simulink library "sm_wheel_loader_lib"  (R2025a)
settings: Solver=VariableStepAuto  StartTime=0.0  StopTime=10.0  RelTol=1e-3
undefined symbols (not defined in the file): AToTOrificeVector, BiPOrificeVector, boomHEArea, boomREArea, BToTOrificeVector, fluids, GRake, GToothL, GToothR, HMPST, HydFcnParams, logLoad, Position, PToAOrificeVector, PToBOrificeVector, RakeL, RakeR, testInput, Wheel_Loader, X, Y, Z
libraries: sm_lib x694, fl_lib x183, nesl_utility x74, SimscapeFluids_lib x62, sdl_lib x25, cvt_components_lib x25, simulink_extras x5, $bdroot x4, wheel_loader_contact_lib x4, ee_lib x2, SignalEditorBlockLib x1, batteryecm_lib x1
(part 4 of 26)

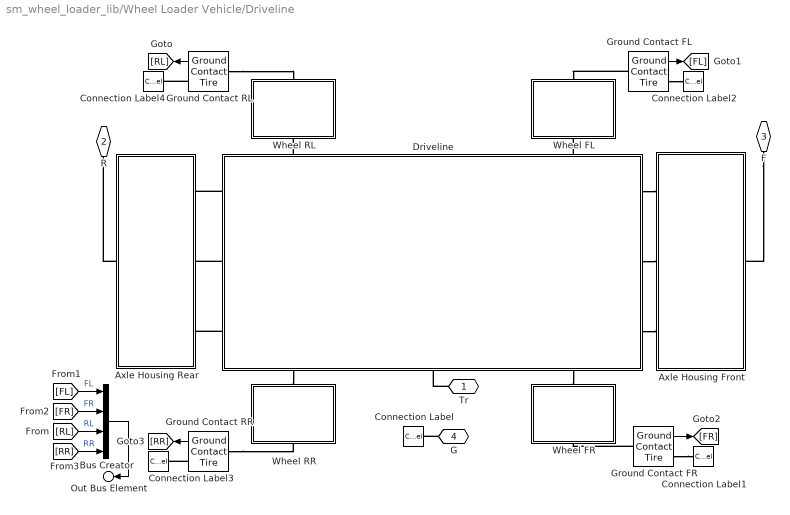
== system sm_wheel_loader_lib/Wheel Loader Vehicle/Driveline ==
  Axle Housing Front : Subsystem  Tag=26328293-4415-CB41-A9FB-B9AA4EE664BB  mask{fa_casing_opc=HMPST.Vis.FAxleHou.opc}
      mask prompts: fa_casing_opc "Casing Opacity"
      mask Display: image('sm_wheel_loader_Driveline3D_FAxleHou_IMAGE.png')
  Axle Housing Rear : Subsystem  Tag=1D918CE5-F562-3F48-9394-464191D609BF  mask{ra_casing_opc=HMPST.Vis.RAxleHou.opc}
      mask prompts: ra_casing_opc "Casing Opacity (0-1)"
      mask Display: image('sm_wheel_loader_Driveline3D_RAxleHou_IMAGE.png')
  Bus Creator : BusCreator  Inputs=4
  Connection Label{,1..4} (5 alike) : ConnectionLabel  Label=G
  Driveline : Subsystem  Variant=on  VariantControlMode=label  VariantControl=Choice  LabelModeActiveChoice=Driveline_1D  mask{popup_driveJointF=CV Joint, popup_driveJointR=CV Joint}
      mask prompts: popup_driveJointF "Driveshaft Joint (front)"; popup_driveJointR "Driveshaft Joint (rear)"
      mask init:
      | if(strcmp(get_param(gcb,'popup_driveJointF'),'CV Joint'))
      |     set_param([gcb '/Driveline 3D'],'popup_driveJointF','CV Joint')
      | else
      |     set_param([gcb '/Driveline 3D'],'popup_driveJointF','U Joint')
      | end
      | if(strcmp(get_param(gcb,'popup_driveJointR'),'CV Joint'))
      |     set_param([gcb '/Driveline 3D'],'popup_driveJointR','CV Joint')
      | else
      |     set_param([gcb '/Driveline 3D'],'popup_driveJointR','U Joint')
      | end
      settings: AttributesFormatString=%<LabelModeActiveChoice>  PortSchema="{\"entries\":[{\"content\":{\"sides\":[{\"content\":{\"connectorIds\":[\"LConn1\",\"LConn2\",\"LConn3\"]},\"type\":\"ConnectorPlacement.EquallySpacedRectSide\",\"uuid\":\"ac94f403-7500-4d3b-9e0f-075c8f20a849\"},{\"content\":{\"connectorIds\":[\"RConn1\",\"RConn2\",\"RConn3\"],\"side\":\"RIGHT\"},\"type\":\"ConnectorPlacement.EquallySpacedRectSide\",\"uuid\":\"0eb844aa-00af-4edc-a570-50ab4e6b66c2\"},{\"content\":{\"connectorIds\":[\"LConn4\",\"LConn5\",\"LConn6\"],\"side\":\"TOP\"},\"type\":\"ConnectorPlacement.EquallySpacedRectSide\",\"uuid\":\"abddfcb0-9899-4667-9404-ac15e4716921\"},{\"content\":{\"connectorIds\":[\"RConn4\",\"RConn5\",\"RConn6\"],\"side\":\"BOTTOM\"},\"type\":\"ConnectorPlacement.EquallySpacedRectSide\",\"uuid\":\"a33fa760-6818-409d-ace3-b40bc7e3acff\"}]},\"type\":\"ConnectorPlacement.EquallySpacedConnector\",\"uuid\":\"2bc03850-1261-46ce-b9b6-2dbda85e9fb0\"}],\"packageUris\":[\"http://schema.mathworks.com/mf0/Connector/R2020b\"],\"version\":\"1.0\"}"
      mask TypeOptions popup_driveJointF: CV Joint | U Joint
      mask TypeOptions popup_driveJointR: CV Joint | U Joint
  Ground Contact FL : wheel_loader_contact_lib/Ground Contact Tire  VariantControl=Choice  LabelModeActiveChoice=Sphere  popup_contact=Sphere  ptcld_xyz=HMPST.Tire.ptcld.FL
  Ground Contact FR : wheel_loader_contact_lib/Ground Contact Tire  VariantControl=Choice  LabelModeActiveChoice=Sphere  popup_contact=Sphere  ptcld_xyz=HMPST.Tire.ptcld.FR
  Ground Contact RL : wheel_loader_contact_lib/Ground Contact Tire  VariantControl=Choice  LabelModeActiveChoice=Sphere  popup_contact=Sphere  ptcld_xyz=HMPST.Tire.ptcld.RL
  Ground Contact RR : wheel_loader_contact_lib/Ground Contact Tire  VariantControl=Choice  LabelModeActiveChoice=Sphere  popup_contact=Sphere  ptcld_xyz=HMPST.Tire.ptcld.RR
  Wheel FL : Subsystem
      mask Display: image('sm_wheel_loader_vehicle_Wheel_IMAGE.png');
  Wheel FR : Subsystem
      mask Display: image('sm_wheel_loader_vehicle_Wheel_IMAGE.png')
  Wheel RL : Subsystem
      mask Display: image('sm_wheel_loader_vehicle_Wheel_IMAGE.png')
  Wheel RR : Subsystem
      mask Display: image('sm_wheel_loader_vehicle_Wheel_IMAGE.png')
  Tr : PMIOPort  Side=Right
  R : PMIOPort  Port=2  Side=Right
  F : PMIOPort  Port=3  Side=Right
  G : PMIOPort  Port=4  Side=Right
  Out Bus Element : Outport  PortName=m  Element=Wheel
  wires:
  Bus Creator/1 -> Out Bus Element/1
  [RR] -> Bus Creator/4  "RR"
  [RL] -> Bus Creator/3  "RL"
  [FR] -> Bus Creator/2  "FR"
  [FL] -> Bus Creator/1  "FL"
  Ground Contact RR/1 -> [RR]
  Ground Contact FR/1 -> [FR]
  Ground Contact FL/1 -> [FL]
  Ground Contact RL/1 -> [RL]
  connections:
  Tr/RConn1 -- Driveline/RConn2
  Ground Contact RL/RConn1 -- Connection Label4/LConn1
  Ground Contact RL/LConn1 -- Wheel RL/LConn1
  Ground Contact RR/RConn1 -- Connection Label3/LConn1
  Ground Contact FL/RConn1 -- Connection Label2/LConn1
  Ground Contact FR/RConn1 -- Connection Label1/LConn1
  G/RConn1 -- Connection Label/LConn1
  Ground Contact FR/LConn1 -- Wheel FR/RConn1
  Driveline/RConn3 -- Wheel FR/LConn1
  Driveline/LConn3 -- Wheel FL/RConn1
  Ground Contact FL/LConn1 -- Wheel FL/LConn1
  Driveline/LConn1 -- Wheel RL/RConn1
  Ground Contact RR/LConn1 -- Wheel RR/RConn1
  Driveline/RConn1 -- Wheel RR/LConn1
  Driveline/RConn6 -- Axle Housing Front/LConn3
  Driveline/RConn5 -- Axle Housing Front/LConn2
  Driveline/RConn4 -- Axle Housing Front/LConn1
  Driveline/LConn6 -- Axle Housing Rear/RConn3
  Driveline/LConn5 -- Axle Housing Rear/RConn2
  Driveline/LConn4 -- Axle Housing Rear/RConn1
  F/RConn1 -- Axle Housing Front/RConn1
  Axle Housing Rear/LConn1 -- R/RConn1

== system sm_wheel_loader_lib/Wheel Loader Vehicle/Frame Front ==
  Camera Frames : Subsystem
  Fender FL : Subsystem  Tag=23FC4218-D579-E34B-A76B-8575254F2127
  Fender FR : Subsystem  Tag=09759EF1-6615-2140-AB69-C7D1A2E7CB45
  FrontFrame : Subsystem  Tag=8DD4DE4B-D0E2-8341-9F65-F61D78DC0BCD
  Lights : Subsystem
  SteeringActRodBearing : Subsystem  Tag=03D27E01-1F06-D945-BD84-AA4BCEEC5D59
  Transform Lights : sm_lib/Frames and Transforms/Rigid Transform  RotationMethod=None  FollAlignAxisA=+X  BaseAlignAxisA=+Y  FollAlignAxisB=+Y  BaseAlignAxisB=+Z  RotationStandardAxis=+Z  RotationAngle=0.0  RotationAngleUnits=deg  RotationArbitraryAxis=[0 0 1]  RotationSequenceAxes=FollowerAxes  RotationSequence=XYX  RotationSequenceAngles=[0 0 0]  RotationSequenceAnglesUnits=deg  RotationMatrix=[1 0 0; 0 1 0; 0 0 1]  Quaternion=[1 0 0 0]  TranslationMethod=Cartesian  TranslationCartesianOffset=[0 0 -0.1895]  TranslationCartesianOffsetUnits=m  TranslationStandardAxis=+Z  TranslationStandardOffset=0  TranslationStandardOffsetUnits=m  TranslationROffset=0  TranslationROffsetUnits=m  TranslationThetaOffset=0  TranslationThetaOffsetUnits=deg  TranslationZOffset=0  TranslationZOffsetUnits=m
  Transform Ref : sm_lib/Frames and Transforms/Rigid Transform  RotationMethod=StandardAxis  FollAlignAxisA=+X  BaseAlignAxisA=+Y  FollAlignAxisB=+Y  BaseAlignAxisB=+Z  RotationStandardAxis=+Z  RotationAngle=90  RotationAngleUnits=deg  RotationArbitraryAxis=[0 0 1]  RotationSequenceAxes=FollowerAxes  RotationSequence=XYX  RotationSequenceAngles=[0 0 0]  RotationSequenceAnglesUnits=deg  RotationMatrix=[1 0 0; 0 1 0; 0 0 1]  Quaternion=[1 0 0 0]  TranslationMethod=Cartesian  TranslationCartesianOffset=[0 0.8705 -0.69773+0.1143]  TranslationCartesianOffsetUnits=m  TranslationStandardAxis=+Z  TranslationStandardOffset=0  TranslationStandardOffsetUnits=m  TranslationROffset=0  TranslationROffsetUnits=m  TranslationThetaOffset=0  TranslationThetaOffsetUnits=deg  TranslationZOffset=0  TranslationZOffsetUnits=m
  Steer : PMIOPort  Side=Left
  Hinge : PMIOPort  Port=2  Side=Left
  LiftL : PMIOPort  Port=3  Side=Right
  LiftR : PMIOPort  Port=4  Side=Right
  Tilt : PMIOPort  Port=5  Side=Right
  Arm : PMIOPort  Port=6  Side=Right
  Drive : PMIOPort  Port=7  Side=Left
  Ref : PMIOPort  Port=8  Side=Right
  connections:
  Lights/LConn1 -- Transform Lights/RConn1
  FrontFrame/RConn3 -- LiftR/RConn1
  Steer/RConn1 -- FrontFrame/LConn1
  Fender FL/LConn1 -- FrontFrame/RConn7
  FrontFrame/RConn2 -- LiftL/RConn1
  Fender FR/LConn1 -- FrontFrame/RConn8
  SteeringActRodBearing/LConn1 -- FrontFrame/RConn1
  FrontFrame/RConn6 -- Drive/RConn1
  FrontFrame/RConn5 -- Arm/RConn1
  FrontFrame/RConn4 -- Tilt/RConn1
  Hinge/RConn1 -- Transform Ref/LConn1 -- Camera Frames/LConn1 -- Transform Lights/LConn1 -- FrontFrame/LConn2
  Ref/RConn1 -- Transform Ref/RConn1

== system sm_wheel_loader_lib/Wheel Loader Vehicle/Frame Rear ==
  BusElementIn : Inport  PortName=Cmd
  Bus Selector : BusSelector  OutputSignals=Operator.SteerCmd
  Cab : Subsystem  Tag=8AB14510-8440-2D42-A5EA-732CCF7C6FFF
  Camera Frames : Subsystem
  Chassis : Subsystem  Tag=0034DD1C-3F78-EA48-8EB0-FD1E79A95281
  Counterweight : Subsystem  Tag=99BCECF5-04B2-334D-A294-C62C2B495A17
  Damper Steering : fl_lib/Mechanical/Rotational Elements/Rotational Damper  D=0.001 N*m*s/rad  w_specify=off  w_priority=None  w=0 rad/s  w_nominal_specify=off  w_nominal_value=1  w_nominal_unit=rad/s  t_specify=off  t_priority=None  t=0 N*m  t_nominal_specify=off  t_nominal_value=1  t_nominal_unit=N*m
  Fender RL : Subsystem  Tag=D7356064-A80E-C343-BF50-4E22E2FDD7AB
  Fender RR : Subsystem  Tag=9CFF811C-0389-C14E-A239-3CC5CD817F6B
  Handles Panels : Subsystem
  Hood : Subsystem  Tag=528F8BEE-8CB9-ED45-8BD2-87AC8441592E
  Mechanical Rotational Reference : fl_lib/Mechanical/Rotational Elements/Mechanical Rotational Reference
  Reference Frame : sm_lib/Frames and Transforms/Reference Frame
  Revolute Steer : sm_lib/Joints/Revolute Joint  JointMode=Normal  CompositeWrenchDir=FollowerOnBase  CompositeWrenchFrame=BaseFrame  SenseConstraintForce=off  SenseConstraintTorque=off  SenseTotalForce=off  SenseTotalTorque=off  PositionTargetSpecify=off  PositionTargetPriority=High  PositionTargetValue=0  PositionTargetValueUnits=deg  VelocityTargetSpecify=off  VelocityTargetPriority=High  VelocityTargetValue=0  VelocityTargetValueUnits=deg/s  EquilibriumPosition=0  EquilibriumPositionUnits=deg  SpringStiffness=0  SpringStiffnessUnits=N*m/deg  DampingCoefficient=0  DampingCoefficientUnits=N*m/(deg/s)  LowerLimitSpecify=off  LowerLimitBound=-90  LowerLimitBoundUnits=deg  LowerLimitStiffness=1e4  LowerLimitStiffnessUnits=N*m/deg  LowerLimitDamping=10  LowerLimitDampingUnits=N*m/(deg/s)  LowerLimitTransitionRegionWidth=0.1  LowerLimitTransitionRegionWidthUnits=deg  UpperLimitSpecify=off  UpperLimitBound=90  UpperLimitBoundUnits=deg  UpperLimitStiffness=1e4  UpperLimitStiffnessUnits=N*m/deg  UpperLimitDamping=10  UpperLimitDampingUnits=N*m/(deg/s)  UpperLimitTransitionRegionWidth=0.1  UpperLimitTransitionRegionWidthUnits=deg  TorqueActuationMode=ComputedTorque  MotionActuationMode=InputMotion  SensePosition=off  SenseVelocity=on  SenseAcceleration=off  SenseTorqueForce=off  SenseLowerLimitTorqueForce=off  SenseUpperLimitTorqueForce=off
  Rigid Transform : sm_lib/Frames and Transforms/Rigid Transform  RotationMethod=StandardAxis  FollAlignAxisA=+X  BaseAlignAxisA=+Y  FollAlignAxisB=+Y  BaseAlignAxisB=+Z  RotationStandardAxis=+X  RotationAngle=-25  RotationAngleUnits=deg  RotationArbitraryAxis=[0 0 1]  RotationSequenceAxes=FollowerAxes  RotationSequence=XYX  RotationSequenceAngles=[0 0 0]  RotationSequenceAnglesUnits=deg  RotationMatrix=[1 0 0;0 1 0;0 0 1]  Quaternion=[1 0 0 0]  TranslationMethod=Cartesian  TranslationCartesianOffset=[0 0.25 0.45]  TranslationCartesianOffsetUnits=m  TranslationStandardAxis=+Z  TranslationStandardOffset=0  TranslationStandardOffsetUnits=m  TranslationROffset=0  TranslationROffsetUnits=m  TranslationThetaOffset=0  TranslationThetaOffsetUnits=deg  TranslationZOffset=0  TranslationZOffsetUnits=m
  Simulink-PS Converter : nesl_utility/Simulink-PS Converter  PhysicalDomain=network_engine_domain  SubClassName=ps_input  LeftPortType=input  RightPortType=output  PseudoPeriodic=off  Frequencies=[]  NoiseDistribution=none  NoiseParameters=[]  Unit=rad  AffineConversion=off  FilteringAndDerivatives=filter  SimscapeFilterOrder=2  InputFilterTimeConstant=0.01  UdotUserProvided=0
  Steering Wheel : Subsystem
  SteeringActCylBearing : Subsystem  Tag=3B841C06-DAE6-6448-91C4-4496AD0D8B5F
  SteeringCoupler : Subsystem  Tag=2E9E311A-265F-DD4B-8FE4-6B9B9F7FC7AE
  Transform Handles : sm_lib/Frames and Transforms/Rigid Transform  RotationMethod=None  FollAlignAxisA=+X  BaseAlignAxisA=+Y  FollAlignAxisB=+Y  BaseAlignAxisB=+Z  RotationStandardAxis=+Z  RotationAngle=0.0  RotationAngleUnits=deg  RotationArbitraryAxis=[0 0 1]  RotationSequenceAxes=FollowerAxes  RotationSequence=XYX  RotationSequenceAngles=[0 0 0]  RotationSequenceAnglesUnits=deg  RotationMatrix=[1 0 0; 0 1 0; 0 0 1]  Quaternion=[1 0 0 0]  TranslationMethod=Cartesian  TranslationCartesianOffset=[0 0 -0.1895]  TranslationCartesianOffsetUnits=m  TranslationStandardAxis=+Z  TranslationStandardOffset=0  TranslationStandardOffsetUnits=m  TranslationROffset=0  TranslationROffsetUnits=m  TranslationThetaOffset=0  TranslationThetaOffsetUnits=deg  TranslationZOffset=0  TranslationZOffsetUnits=m
  Velocity Source Steering Wheel : fl_lib/Mechanical/Mechanical Sources/Ideal Angular Velocity Source
  Steer : PMIOPort  Side=Right
  Hinge : PMIOPort  Port=2  Side=Right
  Drive : PMIOPort  Port=3  Side=Right
  S : PMIOPort  Port=4  Side=Left
  wires:
  BusElementIn/1 -> Bus Selector/1
  Bus Selector/1 -> Simulink-PS Converter/1  "<SteerCmd>"
  connections:
  Handles Panels/LConn1 -- Transform Handles/RConn1
  Hinge/RConn1 -- Transform Handles/LConn1 -- Camera Frames/LConn1 -- Chassis/RConn4
  Chassis/RConn2 -- SteeringActCylBearing/LConn1
  Cab/RConn1 -- Hood/LConn1
  SteeringCoupler/LConn1 -- Chassis/RConn3
  Cab/LConn1 -- Chassis/RConn5
  Reference Frame/RConn1 -- Chassis/LConn1
  Chassis/RConn8 -- Fender RR/LConn1
  Chassis/RConn9 -- Fender RL/LConn1
  Counterweight/LConn1 -- Chassis/RConn6
  Chassis/RConn7 -- Drive/RConn1
  Chassis/RConn1 -- Steer/RConn1
  Rigid Transform/LConn1 -- Cab/RConn2
  Revolute Steer/LConn1 -- Rigid Transform/RConn1
  Revolute Steer/RConn1 -- Steering Wheel/LConn1
  Simulink-PS Converter/RConn1 -- Revolute Steer/LConn2
  Revolute Steer/RConn2 -- Velocity Source Steering Wheel/RConn1
  Damper Steering/RConn1 -- Velocity Source Steering Wheel/RConn2 -- Mechanical Rotational Reference/LConn1
  Velocity Source Steering Wheel/LConn1 -- S/RConn1 -- Damper Steering/LConn1

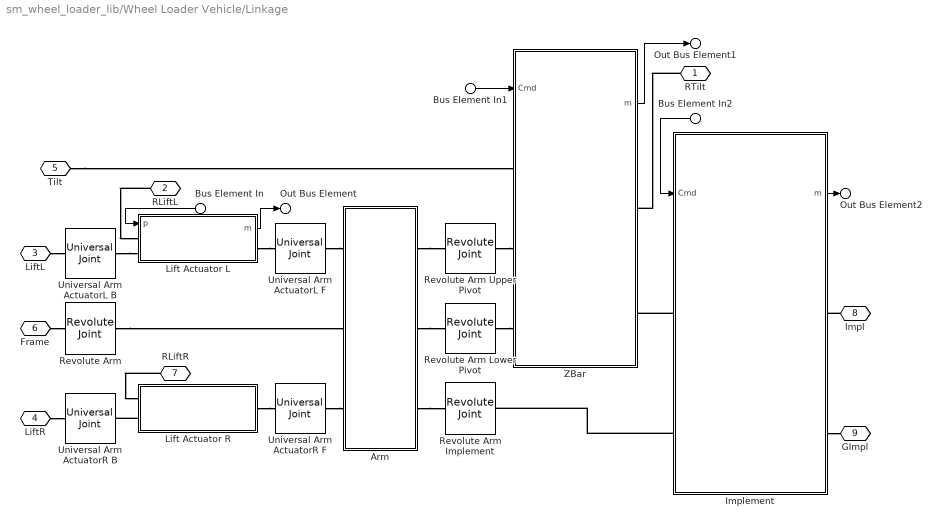
== system sm_wheel_loader_lib/Wheel Loader Vehicle/Linkage ==
  Bus Element In : Inport  PortName=Cmd
  Bus Element In1 : Inport  PortName=Cmd
  Bus Element In2 : Inport  PortName=Cmd
  Arm : Subsystem  Tag=09C7D6F6-616B-0C44-9F51-2EB55AEC562F
      mask Display: image('sm_wheel_loader_vehicle_linkage_Arm_IMAGE.png')
  Implement : Subsystem  Variant=on  VariantControlMode=label  VariantControl=Choice  LabelModeActiveChoice=Bucket  mask{popup_actuator_model=Position}
      mask prompts: popup_actuator_model "Actuator Mode"
      mask init:
      | if(strcmp(get_param(gcb,'popup_actuator_model'),'Shaft'))
      |     set_param([gcb '/Grapple'],'popup_actuator_model','Shaft')
      | else
      |     set_param([gcb '/Grapple'],'popup_actuator_model','Position')
      | end
      settings: AttributesFormatString=%<LabelModeActiveChoice>
      mask TypeOptions popup_actuator_model: Shaft | Position
  Lift Actuator L : Subsystem  Tag=a4be8fe8-02aa-459b-b2da-d5d2a08e5d74  mask{popup_actuator_model=Position}
      mask prompts: popup_actuator_model "Actuator Mode"
      mask init:
      | if(strcmp(get_param(gcb,'popup_actuator_model'),'Shaft'))
      |     set_param([gcb '/Actuator'],'LabelModeActiveChoice','Shaft')
      | else
      |     set_param([gcb '/Actuator'],'LabelModeActiveChoice','Position')
      | end
      mask TypeOptions popup_actuator_model: Shaft | Position
      mask Display:
      | if(strcmp(get_param(gcb,'popup_actuator_model'),'Position'))
      |     image('sm_wheel_loader_actuator_intfPosition_IMAGE.png')
      | else
      |     image('sm_wheel_loader_actuator_intfShaft_IMAGE.png')
      | end
  Lift Actuator R : Subsystem  mask{popup_actuator_model=Position}
      mask prompts: popup_actuator_model "Actuator Mode"
      mask init:
      | if(strcmp(get_param(gcb,'popup_actuator_model'),'Shaft'))
      |     set_param([gcb '/Actuator'],'LabelModeActiveChoice','Shaft')
      | else
      |     set_param([gcb '/Actuator'],'LabelModeActiveChoice','Position')
      | end
      mask TypeOptions popup_actuator_model: Shaft | Position
      mask Display:
      | if(strcmp(get_param(gcb,'popup_actuator_model'),'Position'))
      |     image('sm_wheel_loader_actuator_para_intfNone_IMAGE.png')
      | else
      |     image('sm_wheel_loader_actuator_para_intfShaft_IMAGE.png')
      | end
  Revolute Arm : sm_lib/Joints/Revolute Joint  JointMode=Normal  CompositeWrenchDir=FollowerOnBase  CompositeWrenchFrame=BaseFrame  SenseConstraintForce=off  SenseConstraintTorque=off  SenseTotalForce=off  SenseTotalTorque=off  PositionTargetSpecify=off  PositionTargetPriority=High  PositionTargetValue=0  PositionTargetValueUnits=deg  VelocityTargetSpecify=off  VelocityTargetPriority=High  VelocityTargetValue=0  VelocityTargetValueUnits=deg/s  EquilibriumPosition=0  EquilibriumPositionUnits=deg  SpringStiffness=0  SpringStiffnessUnits=N*m/deg  DampingCoefficient=0  DampingCoefficientUnits=N*m/(rad/s)  LowerLimitSpecify=off  LowerLimitBound=-90  LowerLimitBoundUnits=deg  LowerLimitStiffness=1e4  LowerLimitStiffnessUnits=N*m/deg  LowerLimitDamping=10  LowerLimitDampingUnits=N*m/(deg/s)  LowerLimitTransitionRegionWidth=0.1  LowerLimitTransitionRegionWidthUnits=deg  UpperLimitSpecify=off  UpperLimitBound=90  UpperLimitBoundUnits=deg  UpperLimitStiffness=1e4  UpperLimitStiffnessUnits=N*m/deg  UpperLimitDamping=10  UpperLimitDampingUnits=N*m/(deg/s)  UpperLimitTransitionRegionWidth=0.1  UpperLimitTransitionRegionWidthUnits=deg  TorqueActuationMode=NoTorque  MotionActuationMode=ComputedMotion  SensePosition=off  SenseVelocity=off  SenseAcceleration=off  SenseTorqueForce=off  SenseLowerLimitTorqueForce=off  SenseUpperLimitTorqueForce=off
  Revolute Arm Implement : sm_lib/Joints/Revolute Joint  JointMode=Normal  CompositeWrenchDir=FollowerOnBase  CompositeWrenchFrame=BaseFrame  SenseConstraintForce=off  SenseConstraintTorque=off  SenseTotalForce=off  SenseTotalTorque=off  PositionTargetSpecify=off  PositionTargetPriority=High  PositionTargetValue=0  PositionTargetValueUnits=deg  VelocityTargetSpecify=off  VelocityTargetPriority=High  VelocityTargetValue=0  VelocityTargetValueUnits=deg/s  EquilibriumPosition=0  EquilibriumPositionUnits=deg  SpringStiffness=0  SpringStiffnessUnits=N*m/deg  DampingCoefficient=0  DampingCoefficientUnits=N*m/(deg/s)  LowerLimitSpecify=off  LowerLimitBound=-90  LowerLimitBoundUnits=deg  LowerLimitStiffness=1e4  LowerLimitStiffnessUnits=N*m/deg  LowerLimitDamping=10  LowerLimitDampingUnits=N*m/(deg/s)  LowerLimitTransitionRegionWidth=0.1  LowerLimitTransitionRegionWidthUnits=deg  UpperLimitSpecify=off  UpperLimitBound=90  UpperLimitBoundUnits=deg  UpperLimitStiffness=1e4  UpperLimitStiffnessUnits=N*m/deg  UpperLimitDamping=10  UpperLimitDampingUnits=N*m/(deg/s)  UpperLimitTransitionRegionWidth=0.1  UpperLimitTransitionRegionWidthUnits=deg  TorqueActuationMode=NoTorque  MotionActuationMode=ComputedMotion  SensePosition=off  SenseVelocity=off  SenseAcceleration=off  SenseTorqueForce=off  SenseLowerLimitTorqueForce=off  SenseUpperLimitTorqueForce=off
  Revolute Arm Lower Pivot : sm_lib/Joints/Revolute Joint  JointMode=Normal  CompositeWrenchDir=FollowerOnBase  CompositeWrenchFrame=BaseFrame  SenseConstraintForce=off  SenseConstraintTorque=off  SenseTotalForce=off  SenseTotalTorque=off  PositionTargetSpecify=off  PositionTargetPriority=High  PositionTargetValue=0  PositionTargetValueUnits=deg  VelocityTargetSpecify=off  VelocityTargetPriority=High  VelocityTargetValue=0  VelocityTargetValueUnits=deg/s  EquilibriumPosition=0  EquilibriumPositionUnits=deg  SpringStiffness=0  SpringStiffnessUnits=N*m/deg  DampingCoefficient=0  DampingCoefficientUnits=N*m/(deg/s)  LowerLimitSpecify=off  LowerLimitBound=-90  LowerLimitBoundUnits=deg  LowerLimitStiffness=1e4  LowerLimitStiffnessUnits=N*m/deg  LowerLimitDamping=10  LowerLimitDampingUnits=N*m/(deg/s)  LowerLimitTransitionRegionWidth=0.1  LowerLimitTransitionRegionWidthUnits=deg  UpperLimitSpecify=off  UpperLimitBound=90  UpperLimitBoundUnits=deg  UpperLimitStiffness=1e4  UpperLimitStiffnessUnits=N*m/deg  UpperLimitDamping=10  UpperLimitDampingUnits=N*m/(deg/s)  UpperLimitTransitionRegionWidth=0.1  UpperLimitTransitionRegionWidthUnits=deg  TorqueActuationMode=NoTorque  MotionActuationMode=ComputedMotion  SensePosition=off  SenseVelocity=off  SenseAcceleration=off  SenseTorqueForce=off  SenseLowerLimitTorqueForce=off  SenseUpperLimitTorqueForce=off
  Revolute Arm Upper Pivot : sm_lib/Joints/Revolute Joint  JointMode=Normal  CompositeWrenchDir=FollowerOnBase  CompositeWrenchFrame=BaseFrame  SenseConstraintForce=off  SenseConstraintTorque=off  SenseTotalForce=off  SenseTotalTorque=off  PositionTargetSpecify=off  PositionTargetPriority=High  PositionTargetValue=0  PositionTargetValueUnits=deg  VelocityTargetSpecify=off  VelocityTargetPriority=High  VelocityTargetValue=0  VelocityTargetValueUnits=deg/s  EquilibriumPosition=0  EquilibriumPositionUnits=deg  SpringStiffness=0  SpringStiffnessUnits=N*m/deg  DampingCoefficient=0  DampingCoefficientUnits=N*m/(deg/s)  LowerLimitSpecify=off  LowerLimitBound=-90  LowerLimitBoundUnits=deg  LowerLimitStiffness=1e4  LowerLimitStiffnessUnits=N*m/deg  LowerLimitDamping=10  LowerLimitDampingUnits=N*m/(deg/s)  LowerLimitTransitionRegionWidth=0.1  LowerLimitTransitionRegionWidthUnits=deg  UpperLimitSpecify=off  UpperLimitBound=90  UpperLimitBoundUnits=deg  UpperLimitStiffness=1e4  UpperLimitStiffnessUnits=N*m/deg  UpperLimitDamping=10  UpperLimitDampingUnits=N*m/(deg/s)  UpperLimitTransitionRegionWidth=0.1  UpperLimitTransitionRegionWidthUnits=deg  TorqueActuationMode=NoTorque  MotionActuationMode=ComputedMotion  SensePosition=off  SenseVelocity=off  SenseAcceleration=off  SenseTorqueForce=off  SenseLowerLimitTorqueForce=off  SenseUpperLimitTorqueForce=off
  Universal Arm ActuatorL B : sm_lib/Joints/Universal Joint  JointMode=Normal  CompositeWrenchDir=FollowerOnBase  CompositeWrenchFrame=BaseFrame  SenseConstraintForce=off  SenseConstraintTorque=off  SenseTotalForce=off  SenseTotalTorque=off  RxPositionTargetSpecify=off  RxPositionTargetPriority=High  RxPositionTargetValue=0  RxPositionTargetValueUnits=deg  RxVelocityTargetSpecify=off  RxVelocityTargetPriority=High  RxVelocityTargetValue=0  RxVelocityTargetValueUnits=deg/s  RxEquilibriumPosition=0  RxEquilibriumPositionUnits=deg  RxSpringStiffness=0  RxSpringStiffnessUnits=N*m/deg  RxDampingCoefficient=0  RxDampingCoefficientUnits=N*m/(deg/s)  RxLowerLimitSpecify=off  RxLowerLimitBound=-90  RxLowerLimitBoundUnits=deg  RxLowerLimitStiffness=1e4  RxLowerLimitStiffnessUnits=N*m/deg  RxLowerLimitDamping=10  RxLowerLimitDampingUnits=N*m/(deg/s)  RxLowerLimitTransitionRegionWidth=0.1  RxLowerLimitTransitionRegionWidthUnits=deg  RxUpperLimitSpecify=off  RxUpperLimitBound=90  RxUpperLimitBoundUnits=deg  RxUpperLimitStiffness=1e4  RxUpperLimitStiffnessUnits=N*m/deg  RxUpperLimitDamping=10  RxUpperLimitDampingUnits=N*m/(deg/s)  RxUpperLimitTransitionRegionWidth=0.1  RxUpperLimitTransitionRegionWidthUnits=deg  RxTorqueActuationMode=NoTorque  RxMotionActuationMode=ComputedMotion  RxSensePosition=off  RxSenseVelocity=off  RxSenseAcceleration=off  RxSenseTorqueForce=off  RxSenseLowerLimitTorqueForce=off  RxSenseUpperLimitTorqueForce=off  RyPositionTargetSpecify=off  RyPositionTargetPriority=High  RyPositionTargetValue=0  RyPositionTargetValueUnits=deg  RyVelocityTargetSpecify=off  RyVelocityTargetPriority=High  RyVelocityTargetValue=0  RyVelocityTargetValueUnits=deg/s  RyEquilibriumPosition=0  RyEquilibriumPositionUnits=deg  RySpringStiffness=0  RySpringStiffnessUnits=N*m/deg  RyDampingCoefficient=0  RyDampingCoefficientUnits=N*m/(deg/s)  RyLowerLimitSpecify=off  RyLowerLimitBound=-90  RyLowerLimitBoundUnits=deg  RyLowerLimitStiffness=1e4  RyLowerLimitStiffnessUnits=N*m/deg  RyLowerLimitDamping=10  RyLowerLimitDampingUnits=N*m/(deg/s)  RyLowerLimitTransitionRegionWidth=0.1  RyLowerLimitTransitionRegionWidthUnits=deg  RyUpperLimitSpecify=off  RyUpperLimitBound=90  RyUpperLimitBoundUnits=deg  RyUpperLimitStiffness=1e4  RyUpperLimitStiffnessUnits=N*m/deg  RyUpperLimitDamping=10  RyUpperLimitDampingUnits=N*m/(deg/s)  RyUpperLimitTransitionRegionWidth=0.1  RyUpperLimitTransitionRegionWidthUnits=deg  RyTorqueActuationMode=NoTorque  RyMotionActuationMode=ComputedMotion  RySensePosition=off  RySenseVelocity=off  RySenseAcceleration=off  RySenseTorqueForce=off  RySenseLowerLimitTorqueForce=off  RySenseUpperLimitTorqueForce=off
  Universal Arm ActuatorL F : sm_lib/Joints/Universal Joint  JointMode=Normal  CompositeWrenchDir=FollowerOnBase  CompositeWrenchFrame=BaseFrame  SenseConstraintForce=off  SenseConstraintTorque=off  SenseTotalForce=off  SenseTotalTorque=off  RxPositionTargetSpecify=off  RxPositionTargetPriority=High  RxPositionTargetValue=0  RxPositionTargetValueUnits=deg  RxVelocityTargetSpecify=off  RxVelocityTargetPriority=High  RxVelocityTargetValue=0  RxVelocityTargetValueUnits=deg/s  RxEquilibriumPosition=0  RxEquilibriumPositionUnits=deg  RxSpringStiffness=0  RxSpringStiffnessUnits=N*m/deg  RxDampingCoefficient=0  RxDampingCoefficientUnits=N*m/(deg/s)  RxLowerLimitSpecify=off  RxLowerLimitBound=-90  RxLowerLimitBoundUnits=deg  RxLowerLimitStiffness=1e4  RxLowerLimitStiffnessUnits=N*m/deg  RxLowerLimitDamping=10  RxLowerLimitDampingUnits=N*m/(deg/s)  RxLowerLimitTransitionRegionWidth=0.1  RxLowerLimitTransitionRegionWidthUnits=deg  RxUpperLimitSpecify=off  RxUpperLimitBound=90  RxUpperLimitBoundUnits=deg  RxUpperLimitStiffness=1e4  RxUpperLimitStiffnessUnits=N*m/deg  RxUpperLimitDamping=10  RxUpperLimitDampingUnits=N*m/(deg/s)  RxUpperLimitTransitionRegionWidth=0.1  RxUpperLimitTransitionRegionWidthUnits=deg  RxTorqueActuationMode=NoTorque  RxMotionActuationMode=ComputedMotion  RxSensePosition=off  RxSenseVelocity=off  RxSenseAcceleration=off  RxSenseTorqueForce=off  RxSenseLowerLimitTorqueForce=off  RxSenseUpperLimitTorqueForce=off  RyPositionTargetSpecify=off  RyPositionTargetPriority=High  RyPositionTargetValue=0  RyPositionTargetValueUnits=deg  RyVelocityTargetSpecify=off  RyVelocityTargetPriority=High  RyVelocityTargetValue=0  RyVelocityTargetValueUnits=deg/s  RyEquilibriumPosition=0  RyEquilibriumPositionUnits=deg  RySpringStiffness=0  RySpringStiffnessUnits=N*m/deg  RyDampingCoefficient=0  RyDampingCoefficientUnits=N*m/(deg/s)  RyLowerLimitSpecify=off  RyLowerLimitBound=-90  RyLowerLimitBoundUnits=deg  RyLowerLimitStiffness=1e4  RyLowerLimitStiffnessUnits=N*m/deg  RyLowerLimitDamping=10  RyLowerLimitDampingUnits=N*m/(deg/s)  RyLowerLimitTransitionRegionWidth=0.1  RyLowerLimitTransitionRegionWidthUnits=deg  RyUpperLimitSpecify=off  RyUpperLimitBound=90  RyUpperLimitBoundUnits=deg  RyUpperLimitStiffness=1e4  RyUpperLimitStiffnessUnits=N*m/deg  RyUpperLimitDamping=10  RyUpperLimitDampingUnits=N*m/(deg/s)  RyUpperLimitTransitionRegionWidth=0.1  RyUpperLimitTransitionRegionWidthUnits=deg  RyTorqueActuationMode=NoTorque  RyMotionActuationMode=ComputedMotion  RySensePosition=off  RySenseVelocity=off  RySenseAcceleration=off  RySenseTorqueForce=off  RySenseLowerLimitTorqueForce=off  RySenseUpperLimitTorqueForce=off
  Universal Arm ActuatorR B : sm_lib/Joints/Universal Joint  JointMode=Normal  CompositeWrenchDir=FollowerOnBase  CompositeWrenchFrame=BaseFrame  SenseConstraintForce=off  SenseConstraintTorque=off  SenseTotalForce=off  SenseTotalTorque=off  RxPositionTargetSpecify=off  RxPositionTargetPriority=High  RxPositionTargetValue=0  RxPositionTargetValueUnits=deg  RxVelocityTargetSpecify=off  RxVelocityTargetPriority=High  RxVelocityTargetValue=0  RxVelocityTargetValueUnits=deg/s  RxEquilibriumPosition=0  RxEquilibriumPositionUnits=deg  RxSpringStiffness=0  RxSpringStiffnessUnits=N*m/deg  RxDampingCoefficient=0  RxDampingCoefficientUnits=N*m/(deg/s)  RxLowerLimitSpecify=off  RxLowerLimitBound=-90  RxLowerLimitBoundUnits=deg  RxLowerLimitStiffness=1e4  RxLowerLimitStiffnessUnits=N*m/deg  RxLowerLimitDamping=10  RxLowerLimitDampingUnits=N*m/(deg/s)  RxLowerLimitTransitionRegionWidth=0.1  RxLowerLimitTransitionRegionWidthUnits=deg  RxUpperLimitSpecify=off  RxUpperLimitBound=90  RxUpperLimitBoundUnits=deg  RxUpperLimitStiffness=1e4  RxUpperLimitStiffnessUnits=N*m/deg  RxUpperLimitDamping=10  RxUpperLimitDampingUnits=N*m/(deg/s)  RxUpperLimitTransitionRegionWidth=0.1  RxUpperLimitTransitionRegionWidthUnits=deg  RxTorqueActuationMode=NoTorque  RxMotionActuationMode=ComputedMotion  RxSensePosition=off  RxSenseVelocity=off  RxSenseAcceleration=off  RxSenseTorqueForce=off  RxSenseLowerLimitTorqueForce=off  RxSenseUpperLimitTorqueForce=off  RyPositionTargetSpecify=off  RyPositionTargetPriority=High  RyPositionTargetValue=0  RyPositionTargetValueUnits=deg  RyVelocityTargetSpecify=off  RyVelocityTargetPriority=High  RyVelocityTargetValue=0  RyVelocityTargetValueUnits=deg/s  RyEquilibriumPosition=0  RyEquilibriumPositionUnits=deg  RySpringStiffness=0  RySpringStiffnessUnits=N*m/deg  RyDampingCoefficient=0  RyDampingCoefficientUnits=N*m/(deg/s)  RyLowerLimitSpecify=off  RyLowerLimitBound=-90  RyLowerLimitBoundUnits=deg  RyLowerLimitStiffness=1e4  RyLowerLimitStiffnessUnits=N*m/deg  RyLowerLimitDamping=10  RyLowerLimitDampingUnits=N*m/(deg/s)  RyLowerLimitTransitionRegionWidth=0.1  RyLowerLimitTransitionRegionWidthUnits=deg  RyUpperLimitSpecify=off  RyUpperLimitBound=90  RyUpperLimitBoundUnits=deg  RyUpperLimitStiffness=1e4  RyUpperLimitStiffnessUnits=N*m/deg  RyUpperLimitDamping=10  RyUpperLimitDampingUnits=N*m/(deg/s)  RyUpperLimitTransitionRegionWidth=0.1  RyUpperLimitTransitionRegionWidthUnits=deg  RyTorqueActuationMode=NoTorque  RyMotionActuationMode=ComputedMotion  RySensePosition=off  RySenseVelocity=off  RySenseAcceleration=off  RySenseTorqueForce=off  RySenseLowerLimitTorqueForce=off  RySenseUpperLimitTorqueForce=off
  Universal Arm ActuatorR F : sm_lib/Joints/Universal Joint  JointMode=Normal  CompositeWrenchDir=FollowerOnBase  CompositeWrenchFrame=BaseFrame  SenseConstraintForce=off  SenseConstraintTorque=off  SenseTotalForce=off  SenseTotalTorque=off  RxPositionTargetSpecify=off  RxPositionTargetPriority=High  RxPositionTargetValue=0  RxPositionTargetValueUnits=deg  RxVelocityTargetSpecify=off  RxVelocityTargetPriority=High  RxVelocityTargetValue=0  RxVelocityTargetValueUnits=deg/s  RxEquilibriumPosition=0  RxEquilibriumPositionUnits=deg  RxSpringStiffness=0  RxSpringStiffnessUnits=N*m/deg  RxDampingCoefficient=0  RxDampingCoefficientUnits=N*m/(deg/s)  RxLowerLimitSpecify=off  RxLowerLimitBound=-90  RxLowerLimitBoundUnits=deg  RxLowerLimitStiffness=1e4  RxLowerLimitStiffnessUnits=N*m/deg  RxLowerLimitDamping=10  RxLowerLimitDampingUnits=N*m/(deg/s)  RxLowerLimitTransitionRegionWidth=0.1  RxLowerLimitTransitionRegionWidthUnits=deg  RxUpperLimitSpecify=off  RxUpperLimitBound=90  RxUpperLimitBoundUnits=deg  RxUpperLimitStiffness=1e4  RxUpperLimitStiffnessUnits=N*m/deg  RxUpperLimitDamping=10  RxUpperLimitDampingUnits=N*m/(deg/s)  RxUpperLimitTransitionRegionWidth=0.1  RxUpperLimitTransitionRegionWidthUnits=deg  RxTorqueActuationMode=NoTorque  RxMotionActuationMode=ComputedMotion  RxSensePosition=off  RxSenseVelocity=off  RxSenseAcceleration=off  RxSenseTorqueForce=off  RxSenseLowerLimitTorqueForce=off  RxSenseUpperLimitTorqueForce=off  RyPositionTargetSpecify=off  RyPositionTargetPriority=High  RyPositionTargetValue=0  RyPositionTargetValueUnits=deg  RyVelocityTargetSpecify=off  RyVelocityTargetPriority=High  RyVelocityTargetValue=0  RyVelocityTargetValueUnits=deg/s  RyEquilibriumPosition=0  RyEquilibriumPositionUnits=deg  RySpringStiffness=0  RySpringStiffnessUnits=N*m/deg  RyDampingCoefficient=0  RyDampingCoefficientUnits=N*m/(deg/s)  RyLowerLimitSpecify=off  RyLowerLimitBound=-90  RyLowerLimitBoundUnits=deg  RyLowerLimitStiffness=1e4  RyLowerLimitStiffnessUnits=N*m/deg  RyLowerLimitDamping=10  RyLowerLimitDampingUnits=N*m/(deg/s)  RyLowerLimitTransitionRegionWidth=0.1  RyLowerLimitTransitionRegionWidthUnits=deg  RyUpperLimitSpecify=off  RyUpperLimitBound=90  RyUpperLimitBoundUnits=deg  RyUpperLimitStiffness=1e4  RyUpperLimitStiffnessUnits=N*m/deg  RyUpperLimitDamping=10  RyUpperLimitDampingUnits=N*m/(deg/s)  RyUpperLimitTransitionRegionWidth=0.1  RyUpperLimitTransitionRegionWidthUnits=deg  RyTorqueActuationMode=NoTorque  RyMotionActuationMode=ComputedMotion  RySensePosition=off  RySenseVelocity=off  RySenseAcceleration=off  RySenseTorqueForce=off  RySenseLowerLimitTorqueForce=off  RySenseUpperLimitTorqueForce=off
  ZBar : Subsystem  mask{popup_actuator_model=Position}
      mask prompts: popup_actuator_model "Actuator Mode"
      mask TypeOptions popup_actuator_model: Tilt Actuator/popup_actuator_model
      mask Display: image('sm_wheel_loader_vehicle_linkage_zBar_IMAGE.png')
  RTilt : PMIOPort  Side=Right
  RLiftL : PMIOPort  Port=2  Side=Right
  LiftL : PMIOPort  Port=3  Side=Left
  LiftR : PMIOPort  Port=4  Side=Left
  Tilt : PMIOPort  Port=5  Side=Left
  Frame : PMIOPort  Port=6  Side=Left
  RLiftR : PMIOPort  Port=7  Side=Right
  Impl : PMIOPort  Port=8  Side=Right
  GImpl : PMIOPort  Port=9  Side=Right
  Out Bus Element : Outport  PortName=m  Element=Lift
  Out Bus Element1 : Outport  PortName=m  Element=Tilt
  Out Bus Element2 : Outport  PortName=m  Element=Impl
  wires:
  Implement/1(m) -> Out Bus Element2/1
  ZBar/1(m) -> Out Bus Element1/1
  Lift Actuator L/1(m) -> Out Bus Element/1
  Bus Element In/1 -> Lift Actuator L/1(p)
  Bus Element In1/1 -> ZBar/1(Cmd)
  Bus Element In2/1 -> Implement/1(Cmd)
  connections:
  Implement/RConn2 -- GImpl/RConn1
  Implement/LConn2 -- Revolute Arm Implement/RConn1
  Implement/LConn1 -- ZBar/RConn2
  Revolute Arm Lower Pivot/RConn1 -- ZBar/LConn3
  Revolute Arm Upper Pivot/RConn1 -- ZBar/LConn2
  Tilt/RConn1 -- ZBar/LConn1
  Arm/RConn3 -- Revolute Arm Implement/LConn1
  Frame/RConn1 -- Revolute Arm/LConn1
  Arm/RConn2 -- Revolute Arm Lower Pivot/LConn1
  Arm/RConn1 -- Revolute Arm Upper Pivot/LConn1
  Lift Actuator R/RConn1 -- Universal Arm ActuatorR F/LConn1
  LiftR/RConn1 -- Universal Arm ActuatorR B/LConn1
  Lift Actuator L/RConn1 -- Universal Arm ActuatorL F/LConn1
  LiftL/RConn1 -- Universal Arm ActuatorL B/LConn1
  Revolute Arm/RConn1 -- Arm/LConn2
  Universal Arm ActuatorL F/RConn1 -- Arm/LConn1
  Universal Arm ActuatorR F/RConn1 -- Arm/LConn3
  Lift Actuator R/LConn2 -- Universal Arm ActuatorR B/RConn1
  Universal Arm ActuatorL B/RConn1 -- Lift Actuator L/LConn2
  RTilt/RConn1 -- ZBar/RConn1
  RLiftL/RConn1 -- Lift Actuator L/LConn1
  Impl/RConn1 -- Implement/RConn1
  RLiftR/RConn1 -- Lift Actuator R/LConn1

== system sm_wheel_loader_lib/Wheel Loader Vehicle/Load ==
  Load : Inport
  Inertia : Subsystem  VariantControl=Inertia
      mask Display: image('sm_wheel_loader_load_inertia_IMAGE.png')
  Log : Subsystem  VariantControl=Log  mask{base_location=base_pos, base_orientation=base_ori, bin_location=bin_pos, bin_orientation=bin_ori}
      mask prompts: base_location "Base Location [x y z] (m)"; base_orientation "Base Orientation (deg)"; bin_location "Bin Offset [x y z] (m)"; bin_orientation "Bin Orientation about z (deg)"
      mask TypeOptions base_location: Base/TranslationCartesianOffset
      mask TypeOptions base_orientation: Base/RotationAngle
      mask TypeOptions bin_location: Bin/TranslationCartesianOffset
      mask TypeOptions bin_orientation: Bin/RotationAngle
      mask Display: image('sm_wheel_loader_load_log_IMAGE.png');
  None : Subsystem  VariantControl=None
      mask Display: image('sm_wheel_loader_load_none_IMAGE.png')
  S : PMIOPort  Side=Left
  Im : PMIOPort  Port=2  Side=Left

== system sm_wheel_loader_lib/Wheel Loader Vehicle/Steering Actuator ==
  p : Inport
  Actuator : Subsystem  Variant=on  VariantControlMode=label  VariantControl=Steering Actuator  LabelModeActiveChoice=Position
  Cylinder : Subsystem  Tag=FCF28B6E-431D-8349-BF5E-3EB2C80F968D
      mask Display: image('sm_wheel_loader_actuatorCyl_IMAGE.png')
  Rod : Subsystem  Tag=EF0492E4-495B-C348-9A30-98855C88904F
      mask Display: image('sm_wheel_loader_actuatorPiston_IMAGE.png')
  Universal Steering Front : sm_lib/Joints/Universal Joint  JointMode=Normal  CompositeWrenchDir=FollowerOnBase  CompositeWrenchFrame=BaseFrame  SenseConstraintForce=off  SenseConstraintTorque=off  SenseTotalForce=off  SenseTotalTorque=off  RxPositionTargetSpecify=off  RxPositionTargetPriority=High  RxPositionTargetValue=0  RxPositionTargetValueUnits=deg  RxVelocityTargetSpecify=off  RxVelocityTargetPriority=High  RxVelocityTargetValue=0  RxVelocityTargetValueUnits=deg/s  RxEquilibriumPosition=0  RxEquilibriumPositionUnits=deg  RxSpringStiffness=0  RxSpringStiffnessUnits=N*m/deg  RxDampingCoefficient=0  RxDampingCoefficientUnits=N*m/(deg/s)  RxLowerLimitSpecify=off  RxLowerLimitBound=-90  RxLowerLimitBoundUnits=deg  RxLowerLimitStiffness=1e4  RxLowerLimitStiffnessUnits=N*m/deg  RxLowerLimitDamping=10  RxLowerLimitDampingUnits=N*m/(deg/s)  RxLowerLimitTransitionRegionWidth=0.1  RxLowerLimitTransitionRegionWidthUnits=deg  RxUpperLimitSpecify=off  RxUpperLimitBound=90  RxUpperLimitBoundUnits=deg  RxUpperLimitStiffness=1e4  RxUpperLimitStiffnessUnits=N*m/deg  RxUpperLimitDamping=10  RxUpperLimitDampingUnits=N*m/(deg/s)  RxUpperLimitTransitionRegionWidth=0.1  RxUpperLimitTransitionRegionWidthUnits=deg  RxTorqueActuationMode=NoTorque  RxMotionActuationMode=ComputedMotion  RxSensePosition=off  RxSenseVelocity=off  RxSenseAcceleration=off  RxSenseTorqueForce=off  RxSenseLowerLimitTorqueForce=off  RxSenseUpperLimitTorqueForce=off  RyPositionTargetSpecify=off  RyPositionTargetPriority=High  RyPositionTargetValue=0  RyPositionTargetValueUnits=deg  RyVelocityTargetSpecify=off  RyVelocityTargetPriority=High  RyVelocityTargetValue=0  RyVelocityTargetValueUnits=deg/s  RyEquilibriumPosition=0  RyEquilibriumPositionUnits=deg  RySpringStiffness=0  RySpringStiffnessUnits=N*m/deg  RyDampingCoefficient=0  RyDampingCoefficientUnits=N*m/(deg/s)  RyLowerLimitSpecify=off  RyLowerLimitBound=-90  RyLowerLimitBoundUnits=deg  RyLowerLimitStiffness=1e4  RyLowerLimitStiffnessUnits=N*m/deg  RyLowerLimitDamping=10  RyLowerLimitDampingUnits=N*m/(deg/s)  RyLowerLimitTransitionRegionWidth=0.1  RyLowerLimitTransitionRegionWidthUnits=deg  RyUpperLimitSpecify=off  RyUpperLimitBound=90  RyUpperLimitBoundUnits=deg  RyUpperLimitStiffness=1e4  RyUpperLimitStiffnessUnits=N*m/deg  RyUpperLimitDamping=10  RyUpperLimitDampingUnits=N*m/(deg/s)  RyUpperLimitTransitionRegionWidth=0.1  RyUpperLimitTransitionRegionWidthUnits=deg  RyTorqueActuationMode=NoTorque  RyMotionActuationMode=ComputedMotion  RySensePosition=off  RySenseVelocity=off  RySenseAcceleration=off  RySenseTorqueForce=off  RySenseLowerLimitTorqueForce=off  RySenseUpperLimitTorqueForce=off
  Universal Steering R : sm_lib/Joints/Universal Joint  JointMode=Normal  CompositeWrenchDir=FollowerOnBase  CompositeWrenchFrame=BaseFrame  SenseConstraintForce=off  SenseConstraintTorque=off  SenseTotalForce=off  SenseTotalTorque=off  RxPositionTargetSpecify=off  RxPositionTargetPriority=High  RxPositionTargetValue=0  RxPositionTargetValueUnits=deg  RxVelocityTargetSpecify=off  RxVelocityTargetPriority=High  RxVelocityTargetValue=0  RxVelocityTargetValueUnits=deg/s  RxEquilibriumPosition=0  RxEquilibriumPositionUnits=deg  RxSpringStiffness=0  RxSpringStiffnessUnits=N*m/deg  RxDampingCoefficient=0  RxDampingCoefficientUnits=N*m/(deg/s)  RxLowerLimitSpecify=off  RxLowerLimitBound=-90  RxLowerLimitBoundUnits=deg  RxLowerLimitStiffness=1e4  RxLowerLimitStiffnessUnits=N*m/deg  RxLowerLimitDamping=10  RxLowerLimitDampingUnits=N*m/(deg/s)  RxLowerLimitTransitionRegionWidth=0.1  RxLowerLimitTransitionRegionWidthUnits=deg  RxUpperLimitSpecify=off  RxUpperLimitBound=90  RxUpperLimitBoundUnits=deg  RxUpperLimitStiffness=1e4  RxUpperLimitStiffnessUnits=N*m/deg  RxUpperLimitDamping=10  RxUpperLimitDampingUnits=N*m/(deg/s)  RxUpperLimitTransitionRegionWidth=0.1  RxUpperLimitTransitionRegionWidthUnits=deg  RxTorqueActuationMode=NoTorque  RxMotionActuationMode=ComputedMotion  RxSensePosition=off  RxSenseVelocity=off  RxSenseAcceleration=off  RxSenseTorqueForce=off  RxSenseLowerLimitTorqueForce=off  RxSenseUpperLimitTorqueForce=off  RyPositionTargetSpecify=off  RyPositionTargetPriority=High  RyPositionTargetValue=0  RyPositionTargetValueUnits=deg  RyVelocityTargetSpecify=off  RyVelocityTargetPriority=High  RyVelocityTargetValue=0  RyVelocityTargetValueUnits=deg/s  RyEquilibriumPosition=0  RyEquilibriumPositionUnits=deg  RySpringStiffness=0  RySpringStiffnessUnits=N*m/deg  RyDampingCoefficient=0  RyDampingCoefficientUnits=N*m/(deg/s)  RyLowerLimitSpecify=off  RyLowerLimitBound=-90  RyLowerLimitBoundUnits=deg  RyLowerLimitStiffness=1e4  RyLowerLimitStiffnessUnits=N*m/deg  RyLowerLimitDamping=10  RyLowerLimitDampingUnits=N*m/(deg/s)  RyLowerLimitTransitionRegionWidth=0.1  RyLowerLimitTransitionRegionWidthUnits=deg  RyUpperLimitSpecify=off  RyUpperLimitBound=90  RyUpperLimitBoundUnits=deg  RyUpperLimitStiffness=1e4  RyUpperLimitStiffnessUnits=N*m/deg  RyUpperLimitDamping=10  RyUpperLimitDampingUnits=N*m/(deg/s)  RyUpperLimitTransitionRegionWidth=0.1  RyUpperLimitTransitionRegionWidthUnits=deg  RyTorqueActuationMode=NoTorque  RyMotionActuationMode=ComputedMotion  RySensePosition=off  RySenseVelocity=off  RySenseAcceleration=off  RySenseTorqueForce=off  RySenseLowerLimitTorqueForce=off  RySenseUpperLimitTorqueForce=off
  R : PMIOPort  Side=Left
  F : PMIOPort  Port=2  Side=Right
  B : PMIOPort  Port=3  Side=Left
  m : Outport
  wires:
  Actuator/1(m) -> m/1
  p/1 -> Actuator/1(p)
  connections:
  B/RConn1 -- Universal Steering R/LConn1
  Rod/RConn1 -- Universal Steering Front/LConn1
  Universal Steering R/RConn1 -- Cylinder/LConn1
  Universal Steering Front/RConn1 -- F/RConn1
  Actuator/LConn1 -- R/RConn1
  Actuator/LConn2 -- Cylinder/RConn1
  Actuator/RConn1 -- Rod/LConn1

== system sm_wheel_loader_lib/Wheel Loader Vehicle/Subsystem ==
  Link : Inport
  Str : Inport  Port=2
  Bus Selector : BusSelector  OutputSignals=power
  Bus Selector1 : BusSelector  OutputSignals=Lift.power,Tilt.power,Impl.power
  Sum : Sum  Inputs=++++
  pwr : Outport
  wires:
  Str/1 -> Bus Selector/1
  Bus Selector1/1 -> Sum/1  "<power>"
  Link/1 -> Bus Selector1/1
  Bus Selector/1 -> Sum/4  "<power>"
  Bus Selector1/2 -> Sum/2  "<power>"
  Bus Selector1/3 -> Sum/3  "<power>"
  Sum/1 -> pwr/1

== system sm_wheel_loader_lib/CVT Electrical/Control/Control ==
  wCmd : Inport
  wMeas : Inport  Port=2
  Integrator : Integrator
  Ki : Gain  Gain=HMPST.Control.Ki
  Kp : Gain  Gain=HMPST.Control.Kp
  Sum : Sum  Inputs=+-|
  Sum1 : Sum  Inputs=++|
  Transfer Fcn (with initial states) : simulink_extras/Additional Linear/Transfer Fcn (with initial states)  N=[1]  D="[HMPST.Control.tFilt  1]"  X0=0
  Trq : Outport
  wires:
  Sum/1 -> Transfer Fcn (with initial states)/1
  Sum1/1 -> Trq/1
  Kp/1 -> Sum1/2
  Ki/1 -> Integrator/1
  Integrator/1 -> Sum1/1
  Transfer Fcn (with initial states)/1 -> Ki/1, Kp/1
  wMeas/1 -> Sum/2
  wCmd/1 -> Sum/1

== system sm_wheel_loader_lib/CVT Power Split Hydromechanical/HRB/Subsystem ==
  Hydraulic Pressure Sensor : fl_lib/Isothermal Liquid/Sensors/Pressure Sensor (IL)  pressure_measure=foundation.enum.pressure_measure.difference
      settings: InternalSimscapePortConfiguration="{\"Bottom\":[],\"Left\":[{\"id\":\"A\",\"label\":\"A\",\"type\":\"foundation.isothermal_liquid.isothermal_liquid\"}],\"Right\":[{\"id\":\"B\",\"label\":\"B\",\"type\":\"foundation.isothermal_liquid.isothermal_liquid\"},{\"id\":\"P\",\"label\":\"P\",\"type\":\"output\"}],\"Top\":[]}"
      settings: LibrarySourceBlock=|
      | fl_lib/Hydraulic/Hydraulic Sensors/Hydraulic Pressure
      | Sensor
  Hydraulic Reference1 : fl_lib/Isothermal Liquid/Elements/Reservoir (IL)  reservoir_type=foundation.enum.constant_controlled.constant  pressure_spec=foundation.enum.pressure_spec.atmospheric  reservoir_pressure=0.101325 MPa
      settings: LibrarySourceBlock=fl_lib/Hydraulic/Hydraulic Elements/Hydraulic Reference
  PS-Simulink Converter : nesl_utility/PS-Simulink Converter  PhysicalDomain=network_engine_domain  SubClassName=ps_output  LeftPortType=input  RightPortType=output  PseudoPeriodic=off  Frequencies=[]  VectorFormat=1-D array  Unit=MPa  AffineConversion=off
  A : PMIOPort  Side=Left
  p : Outport
  wires:
  PS-Simulink Converter/1 -> p/1
  connections:
  Hydraulic Pressure Sensor/RConn1 -- Hydraulic Reference1/LConn1
  A/RConn1 -- Hydraulic Pressure Sensor/LConn1
  Hydraulic Pressure Sensor/RConn2 -- PS-Simulink Converter/LConn1

== system sm_wheel_loader_lib/CVT Power Split Hydromechanical/Hydrostatic/Charge Pump ==
  Mechanical Rotational Reference : fl_lib/Mechanical/Rotational Elements/Mechanical Rotational Reference
  Pressure Relief Valve : SimscapeFluids_lib/Isothermal Liquid/Valves & Orifices/Pressure Control Valves/Pressure Relief Valve (IL)  set_pressure_spec=foundation.enum.constant_controlled.constant  opening_spec=fluids.isothermal_liquid.valves_orifices.enum.opening_spec.linear  pressure_spec=fluids.isothermal_liquid.valves_orifices.enum.pressure_control_spec.dp  p_set_gauge=0.1 MPa  p_set_differential=chgPumpChkvPdiff MPa  p_range=chgPumpChkvPrange MPa  area_max=chgPumpChkvAmax m^2  area_leak=chgPumpChkvAleak m^2  p_diff_TLU=[0.2 : 0.2 : 1.2] MPa  p_gauge_TLU=[0.2 : 0.2 : 1.2] MPa  valve_area_TLU=[1e-10, 2e-06, 4e-06, 6e-06, 8e-06, 1e-05] m^2  vol_flow_TLU=[1e-09, 3.6e-05, 8.9e-05, .00015, .00023, .00031] m^3/s  area=inf m^2  Cd=0.64  Re_c=150  smoothing_factor=0.01  pressure_recovery=simscape.enum.onoff.off  opening_dynamics=simscape.enum.onoff.off  tau=0.1 s
      settings: InternalSimscapePortConfiguration="{\"Bottom\":[],\"Left\":[{\"id\":\"A\",\"label\":\"A\",\"type\":\"foundation.isothermal_liquid.isothermal_liquid\"}],\"Right\":[{\"id\":\"B\",\"label\":\"B\",\"type\":\"foundation.isothermal_liquid.isothermal_liquid\"}],\"Top\":[]}"
  Pump : SimscapeFluids_lib/Isothermal Liquid/Pumps & Motors/Fixed-Displacement Pump (IL)  leakage_friction_spec=fluids.isothermal_liquid.pumps_motors.enum.pump_motor_loss_spec.analytical  displacement=chgPumpNomDisp cm^3/rev  omega_nominal=chgPumpNomSpd rpm  p_nominal=chgPumpNomPressGain MPa  vol_eff_nominal=chgPumpNomVolEff  mech_eff_nominal=chgPumpNomMechEff  no_load_torque=0 N*m  p_diff_eff_TLU=[.1, 1, 2] MPa  omega_eff_TLU=[25, 50, 100, 200, 300, 400] rad/s  vol_eff_TLU=[.816, .908, .954, .977, .981, .984; .325, .663, .831, .916, .925, .946; .137, .568, .78, .892, .893, .91]  mech_eff_TLU=[.996, .996, .996, .996, .996, .996; .988, .989, .989, .989, .989, .99; .981, .981, .982, .982, .983, .984]  p_diff_loss_TLU=[.1, 1, 2] MPa  omega_loss_TLU=[25, 50, 100, 200, 300, 400] rad/s  vol_loss_TLU=[.023, .023, .023, .023, .0285, .032; .0844, .0842, .0845, .084, .1125, .108; .1079, .108, .11, .108, .1605, .18] * 1e-3 m^3/s  mech_loss_TLU=[.002, .002, .002, .002, .002, .002; .0607, .0556, .0556, .0556, .0556, .0505; .1937, .1937, .1833, .1833, .1729, .1626] N*m  vol_eff_min=1e-3  vol_eff_max=1  mech_eff_min=1e-3  mech_eff_max=1  pressure_threshold=1e-3 MPa  omega_threshold=10 rad/s  supplied_range_check=simscape.enum.assert.action.none  pump_mode_check=simscape.enum.assert.action.none  pressure_check=simscape.enum.assert.action.none  p_min_valid=0.101325 MPa
      settings: InternalSimscapePortConfiguration="{\"Bottom\":[{\"id\":\"A\",\"label\":\"A\",\"type\":\"foundation.isothermal_liquid.isothermal_liquid\"}],\"Left\":[],\"Right\":[{\"id\":\"R\",\"label\":\"R\",\"type\":\"foundation.mechanical.rotational.rotational\"},{\"id\":\"C\",\"label\":\"C\",\"type\":\"foundation.mechanical.rotational.rotational\"}],\"Top\":[{\"id\":\"B\",\"label\":\"B\",\"type\":\"foundation.isothermal_liquid.isothermal_liquid\"}]}"
  Reservoir (IL) : fl_lib/Isothermal Liquid/Elements/Reservoir (IL)  reservoir_type=foundation.enum.constant_controlled.constant  pressure_spec=foundation.enum.pressure_spec.atmospheric  reservoir_pressure=0.101325 MPa
  Outlet : PMIOPort  Side=Right
  C : PMIOPort  Port=2  Side=Left
  connections:
  C/RConn1 -- Pump/RConn1
  Pump/RConn2 -- Mechanical Rotational Reference/LConn1
  Pump/RConn3 -- Pressure Relief Valve/RConn1 -- Reservoir (IL)/LConn1
  Pressure Relief Valve/LConn1 -- Pump/LConn1 -- Outlet/RConn1
